simulink model "lab_2_2"  (R2023b)
settings: Solver=FixedStepAuto  StartTime=0.0  StopTime=10.0  FixedStep=0.001  RelTol=1e-3
undefined symbols (not defined in the file): g, K, T1, T2
settings Model: Creator=nsukh  LastModifiedBy=nsukh

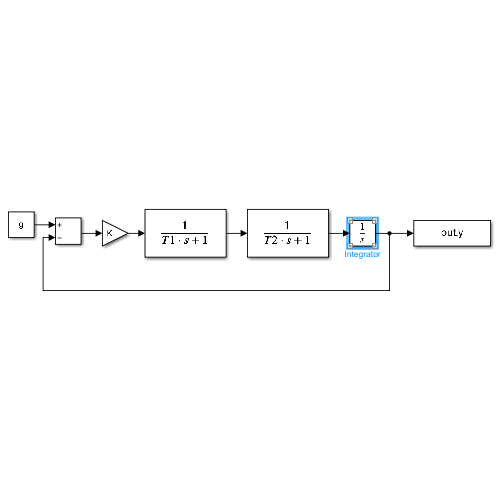
[thumbnail: Simulink's stored preview of the top-level diagram]
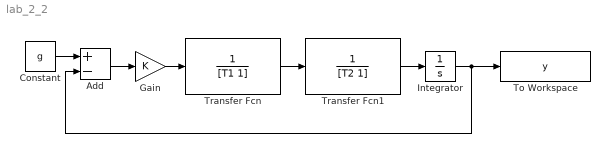
== system lab_2_2 ==
  Add : Sum  Inputs=+-
  Constant : Constant  Value=g  SampleTime=-1
  Gain : Gain  Gain=K
  Integrator : Integrator
  To Workspace : ToWorkspace  VariableName=y  SaveFormat=Timeseries  SampleTime=-1
  Transfer Fcn : TransferFcn  Denominator=[T1 1]
  Transfer Fcn1 : TransferFcn  Denominator=[T2 1]
  wires:
  Transfer Fcn/1 -> Transfer Fcn1/1
  Transfer Fcn1/1 -> Integrator/1
  Gain/1 -> Transfer Fcn/1
  Add/1 -> Gain/1
  Constant/1 -> Add/1
  Integrator/1 -> Add/2, To Workspace/1
